simulink model "Drone_swarm_control"  (R2025a)
settings: Solver=FixedStepAuto  StartTime=0.0  StopTime=180  FixedStep=0.001  RelTol=1e-3
InitFcn:
  | %% Simulation parameters and waypoint trajectory
  | % Initial drone positions.
  | init_0=[0;0;0];
  | d_s=4;
  | init_1=init_0+d_s*[-1.1;0.1;0];
  | init_2=init_0+d_s*[0.3;-1.5;0];
  | init_3=init_0+d_s*[1.6;0.4;0];
  | init_4=init_0+d_s*[0.2;1.8;0];
  | 
  | % Initial battery energy in Wh.
  | E_0=77;
  | gain_2=1;
  | 
  | % PID controller gains.
  | PID_p=20;
  | PID_i=50;
  | PID_d=0;
  | 
  | % Router queues and background traffic.
  | router_buffer=160;
  | router_bandwith=300;
  | router_init_queue=[20,0,0,0,0];
  | traffic_mean=20;
  | traffic_variance=1;
  | 
  | % Communication-rate parameters.
  | F_max=2;
  | F_min=0.5;
  | F_H=(F_max+F_min)/3;
  | P_nc=(1-(F_H-F_min)/F_max);
  | 
  | 
  | % Desired formation offsets.
  | init_f_0=[0;0;0];
  | d_f=10;
  | init_f_1=init_0+d_f*[-1;0;0];
  | init_f_2=init_0+d_f*[0;-1;0];
  | init_f_3=init_0+d_f*[1;0;0];
  | init_f_4=init_0+d_f*[0;1;0];
  | 
  | 
  | % Waypoint mission with a fixed cruise altitude.
  | quota_fissa = -20;
  | 
  | waypoints = [
  |       0   0   0   0;
  |      75   0   quota_fissa   0;
  |     150   0   quota_fissa   0;
  |     225   0   quota_fissa   0;
  |     300   0   quota_fissa   0;
  |     300   0   quota_fissa   0;
  |     225  75   quota_fissa   0;
  |     150 150   quota_fissa   0;
  |      75 225   quota_fissa   0;
  |       0 300   quota_fissa   0;
  |       0 300   quota_fissa   0;
  |      75 300   quota_fissa   0;
  |     150 300   quota_fissa   0;
  |     225 300   quota_fissa   0;
  |     300 300   quota_fissa   0;
  | ... (+79 lines)
undefined symbols (not defined in the file): A_diacenza, DiscIntNeverNeededParam, L
libraries: dspsigops x10, robotcorelib x5, slpidlib x5, dspstat3 x5, simulink x1, uavutilslib x1
(part 2 of 4)

== system Drone_swarm_control/Subsystem1/Subsystem2 ==
  In1 : Inport
  In2 : Inport  Port=2
  In3 : Inport  Port=3
  In4 : Inport  Port=4
  In5 : Inport  Port=5
  Matrix Concatenate1 : Concatenate  NumInputs=5  Mode=Multidimensional array  ConcatenateDimension=2
  Out1 : Outport
  wires:
  In4/1 -> Matrix Concatenate1/4
  In2/1 -> Matrix Concatenate1/2
  In5/1 -> Matrix Concatenate1/5
  Matrix Concatenate1/1 -> Out1/1
  In1/1 -> Matrix Concatenate1/1
  In3/1 -> Matrix Concatenate1/3

== system Drone_swarm_control/Subsystem1/Subsystem3 ==
  In1 : Inport
  In2 : Inport  Port=2
  In3 : Inport  Port=3
  In4 : Inport  Port=4
  In5 : Inport  Port=5
  Matrix Concatenate3 : Concatenate  NumInputs=5  Mode=Multidimensional array  ConcatenateDimension=2
  Out1 : Outport
  wires:
  In5/1 -> Matrix Concatenate3/5
  Matrix Concatenate3/1 -> Out1/1
  In3/1 -> Matrix Concatenate3/3
  In4/1 -> Matrix Concatenate3/4
  In2/1 -> Matrix Concatenate3/2
  In1/1 -> Matrix Concatenate3/1

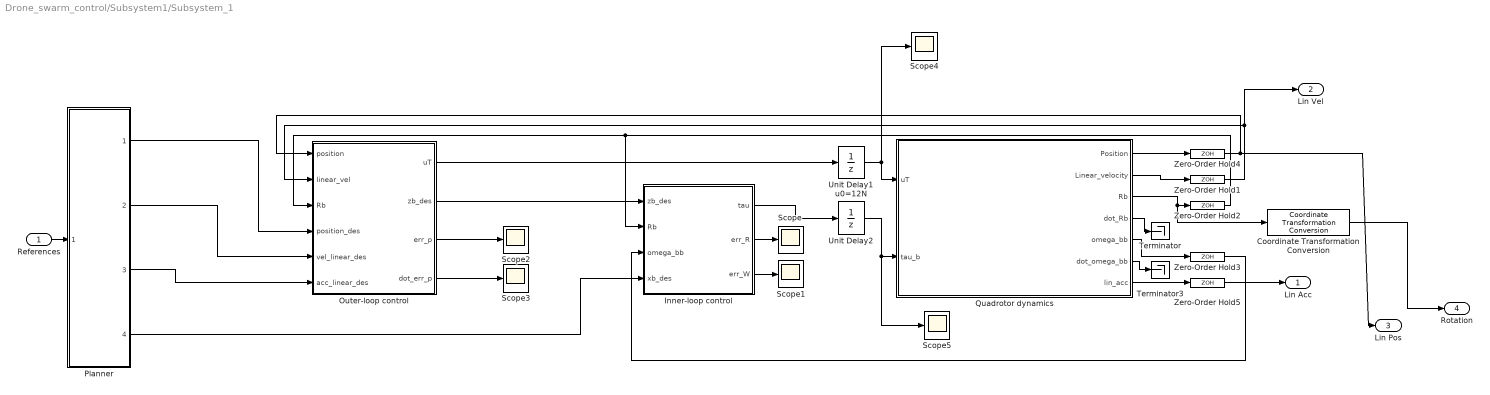
== system Drone_swarm_control/Subsystem1/Subsystem_1 ==
  References : Inport
  Coordinate Transformation Conversion : robotcorelib/Coordinate Transformation Conversion  InputRepresentation=Rotation Matrix  InputEulerSequence=ZYX  ShowTrVecInputPort=on  OutputRepresentation=Quaternion  OutputEulerSequence=ZYX  ShowTrVecOutputPort=on  SimulateUsing=Interpreted execution
  Inner-loop control : Subsystem
  Outer-loop control : MATLAB Function  TreatAsAtomicUnit=on
  Planner : Subsystem
  Quadrotor dynamics : Subsystem
  Scope{,1..5} (6 alike) : Scope
      Scope settings: ActiveDisplayYMinimum=-1.2E-5  ActiveDisplayYMaximum=1.2E-5
      Scope1 settings: ActiveDisplayYMinimum=-1.2E-5  ActiveDisplayYMaximum=1.2E-5
      Scope2 settings: ActiveDisplayYMinimum=-3.9E-5  ActiveDisplayYMaximum=1.1E-5  DataLoggingVariableName=ScopeData2
      Scope3 settings: ActiveDisplayYMinimum=-0.00022  ActiveDisplayYMaximum=0.00011  DataLoggingVariableName=ScopeData3
      Scope4 settings: ActiveDisplayYMinimum=11.66748  ActiveDisplayYMaximum=12.03695  DataLoggingVariableName=ScopeData4
      Scope5 settings: ActiveDisplayYMinimum=-0.02035  ActiveDisplayYMaximum=0.02036  DataLoggingVariableName=ScopeData5
  Terminator : Terminator
  Terminator3 : Terminator
  Unit Delay1 u0=12N : UnitDelay  InitialCondition=12  SampleTime=Ts
  Unit Delay2 : UnitDelay  InitialCondition=[0 0 0]  SampleTime=Ts
  Zero-Order Hold{1..5} (5 alike) : ZeroOrderHold  SampleTime=Ts
  Lin Acc : Outport
  Lin Vel : Outport  Port=2
  Lin Pos : Outport  Port=3
  Rotation : Outport  Port=4
  wires:
  Zero-Order Hold5/1 -> Lin Acc/1
  Quadrotor dynamics/7(lin_acc) -> Zero-Order Hold5/1
  Planner/1(position_des) -> Outer-loop control/4(position_des)
  Quadrotor dynamics/1(Position) -> Zero-Order Hold4/1
  Quadrotor dynamics/3(Rb) -> Zero-Order Hold2/1, Coordinate Transformation Conversion/1
  Quadrotor dynamics/4(dot_Rb) -> Terminator/1
  Planner/4(xb_des) -> Inner-loop control/4(xb_des)
  Inner-loop control/1(tau) -> Unit Delay2/1
  Planner/2(linear_velocity_des) -> Outer-loop control/5(vel_linear_des)
  Quadrotor dynamics/2(Linear_velocity) -> Zero-Order Hold1/1
  Quadrotor dynamics/6(dot_omega_bb) -> Terminator3/1
  Outer-loop control/3(err_p) -> Scope2/1
  Coordinate Transformation Conversion/1 -> Rotation/1
  Quadrotor dynamics/5(omega_bb) -> Zero-Order Hold3/1
  Zero-Order Hold2/1 -> Inner-loop control/2(Rb), Outer-loop control/3(Rb)
  References/1 -> Planner/1(References)
  Planner/3(linear_acceleration_des) -> Outer-loop control/6(acc_linear_des)
  Inner-loop control/3(err_W) -> Scope1/1
  Outer-loop control/2(zb_des) -> Inner-loop control/1(zb_des)
  Inner-loop control/2(err_R) -> Scope/1
  Outer-loop control/1(uT) -> Unit Delay1 u0=12N/1
  Unit Delay2/1 -> Quadrotor dynamics/2(tau_b), Scope5/1
  Zero-Order Hold3/1 -> Inner-loop control/3(omega_bb)
  Unit Delay1 u0=12N/1 -> Scope4/1, Quadrotor dynamics/1(uT)
  Outer-loop control/4(dot_err_p) -> Scope3/1
  Zero-Order Hold1/1 -> Outer-loop control/2(linear_vel), Lin Vel/1
  Zero-Order Hold4/1 -> Outer-loop control/1(position), Lin Pos/1

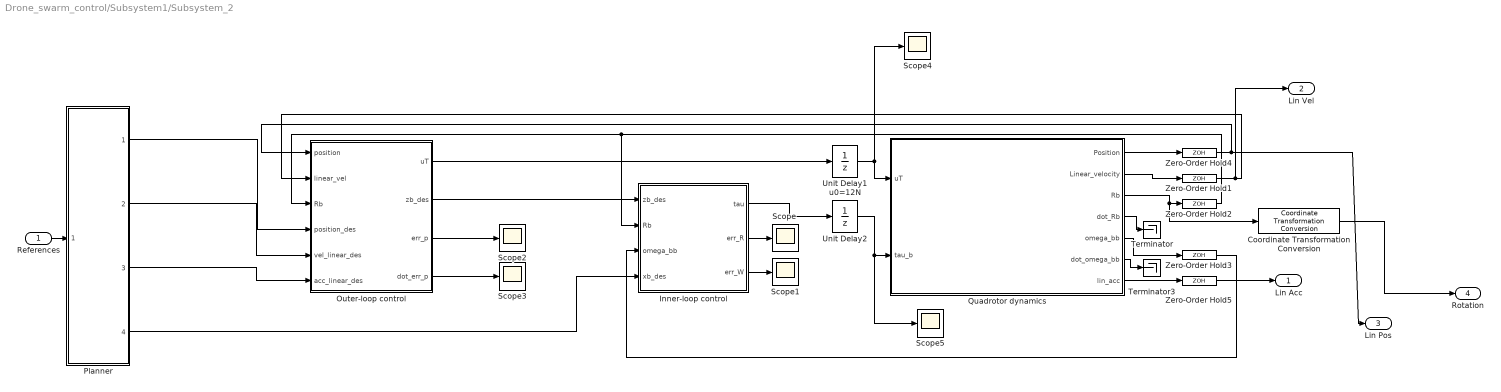
== system Drone_swarm_control/Subsystem1/Subsystem_2 ==
  References : Inport
  Coordinate Transformation Conversion : robotcorelib/Coordinate Transformation Conversion  InputRepresentation=Rotation Matrix  InputEulerSequence=ZYX  ShowTrVecInputPort=on  OutputRepresentation=Quaternion  OutputEulerSequence=ZYX  ShowTrVecOutputPort=on  SimulateUsing=Interpreted execution
  Inner-loop control : Subsystem
  Outer-loop control : MATLAB Function  TreatAsAtomicUnit=on
  Planner : Subsystem
  Quadrotor dynamics : Subsystem
  Scope{,1..5} (6 alike) : Scope
      Scope settings: ActiveDisplayYMinimum=-1.2E-5  ActiveDisplayYMaximum=1.2E-5
      Scope1 settings: ActiveDisplayYMinimum=-1.2E-5  ActiveDisplayYMaximum=1.2E-5
      Scope2 settings: ActiveDisplayYMinimum=-3.9E-5  ActiveDisplayYMaximum=1.1E-5  DataLoggingVariableName=ScopeData2
      Scope3 settings: ActiveDisplayYMinimum=-0.00022  ActiveDisplayYMaximum=0.00011  DataLoggingVariableName=ScopeData3
      Scope4 settings: ActiveDisplayYMinimum=11.66748  ActiveDisplayYMaximum=12.03695  DataLoggingVariableName=ScopeData4
      Scope5 settings: ActiveDisplayYMinimum=-0.02035  ActiveDisplayYMaximum=0.02036  DataLoggingVariableName=ScopeData5
  Terminator : Terminator
  Terminator3 : Terminator
  Unit Delay1 u0=12N : UnitDelay  InitialCondition=12  SampleTime=Ts
  Unit Delay2 : UnitDelay  InitialCondition=[0 0 0]  SampleTime=Ts
  Zero-Order Hold{1..5} (5 alike) : ZeroOrderHold  SampleTime=Ts
  Lin Acc : Outport
  Lin Vel : Outport  Port=2
  Lin Pos : Outport  Port=3
  Rotation : Outport  Port=4
  wires:
  Zero-Order Hold5/1 -> Lin Acc/1
  Quadrotor dynamics/7(lin_acc) -> Zero-Order Hold5/1
  Planner/1(position_des) -> Outer-loop control/4(position_des)
  Quadrotor dynamics/1(Position) -> Zero-Order Hold4/1
  Quadrotor dynamics/3(Rb) -> Zero-Order Hold2/1, Coordinate Transformation Conversion/1
  Quadrotor dynamics/4(dot_Rb) -> Terminator/1
  Planner/4(xb_des) -> Inner-loop control/4(xb_des)
  Inner-loop control/1(tau) -> Unit Delay2/1
  Planner/2(linear_velocity_des) -> Outer-loop control/5(vel_linear_des)
  Quadrotor dynamics/2(Linear_velocity) -> Zero-Order Hold1/1
  Quadrotor dynamics/6(dot_omega_bb) -> Terminator3/1
  Outer-loop control/3(err_p) -> Scope2/1
  Coordinate Transformation Conversion/1 -> Rotation/1
  Quadrotor dynamics/5(omega_bb) -> Zero-Order Hold3/1
  Zero-Order Hold2/1 -> Inner-loop control/2(Rb), Outer-loop control/3(Rb)
  References/1 -> Planner/1(References)
  Planner/3(linear_acceleration_des) -> Outer-loop control/6(acc_linear_des)
  Inner-loop control/3(err_W) -> Scope1/1
  Outer-loop control/2(zb_des) -> Inner-loop control/1(zb_des)
  Inner-loop control/2(err_R) -> Scope/1
  Outer-loop control/1(uT) -> Unit Delay1 u0=12N/1
  Unit Delay2/1 -> Quadrotor dynamics/2(tau_b), Scope5/1
  Zero-Order Hold3/1 -> Inner-loop control/3(omega_bb)
  Unit Delay1 u0=12N/1 -> Scope4/1, Quadrotor dynamics/1(uT)
  Outer-loop control/4(dot_err_p) -> Scope3/1
  Zero-Order Hold1/1 -> Outer-loop control/2(linear_vel), Lin Vel/1
  Zero-Order Hold4/1 -> Outer-loop control/1(position), Lin Pos/1

== system Drone_swarm_control/Subsystem1/Subsystem_3 ==
  References : Inport
  Coordinate Transformation Conversion : robotcorelib/Coordinate Transformation Conversion  InputRepresentation=Rotation Matrix  InputEulerSequence=ZYX  ShowTrVecInputPort=on  OutputRepresentation=Quaternion  OutputEulerSequence=ZYX  ShowTrVecOutputPort=on  SimulateUsing=Interpreted execution
  Inner-loop control : Subsystem
  Outer-loop control : MATLAB Function  TreatAsAtomicUnit=on
  Planner : Subsystem
  Quadrotor dynamics : Subsystem
  Scope{,1..5} (6 alike) : Scope
      Scope settings: ActiveDisplayYMinimum=-1.2E-5  ActiveDisplayYMaximum=1.2E-5
      Scope1 settings: ActiveDisplayYMinimum=-1.2E-5  ActiveDisplayYMaximum=1.2E-5
      Scope2 settings: ActiveDisplayYMinimum=-3.9E-5  ActiveDisplayYMaximum=1.1E-5  DataLoggingVariableName=ScopeData2
      Scope3 settings: ActiveDisplayYMinimum=-0.00022  ActiveDisplayYMaximum=0.00011  DataLoggingVariableName=ScopeData3
      Scope4 settings: ActiveDisplayYMinimum=11.66748  ActiveDisplayYMaximum=12.03695  DataLoggingVariableName=ScopeData4
      Scope5 settings: ActiveDisplayYMinimum=-0.02035  ActiveDisplayYMaximum=0.02036  DataLoggingVariableName=ScopeData5
  Terminator : Terminator
  Terminator3 : Terminator
  Unit Delay1 u0=12N : UnitDelay  InitialCondition=12  SampleTime=Ts
  Unit Delay2 : UnitDelay  InitialCondition=[0 0 0]  SampleTime=Ts
  Zero-Order Hold{1..5} (5 alike) : ZeroOrderHold  SampleTime=Ts
  Lin Acc : Outport
  Lin Vel : Outport  Port=2
  Lin Pos : Outport  Port=3
  Rotation : Outport  Port=4
  wires:
  Zero-Order Hold5/1 -> Lin Acc/1
  Quadrotor dynamics/7(lin_acc) -> Zero-Order Hold5/1
  Planner/1(position_des) -> Outer-loop control/4(position_des)
  Quadrotor dynamics/1(Position) -> Zero-Order Hold4/1
  Quadrotor dynamics/3(Rb) -> Zero-Order Hold2/1, Coordinate Transformation Conversion/1
  Quadrotor dynamics/4(dot_Rb) -> Terminator/1
  Planner/4(xb_des) -> Inner-loop control/4(xb_des)
  Inner-loop control/1(tau) -> Unit Delay2/1
  Planner/2(linear_velocity_des) -> Outer-loop control/5(vel_linear_des)
  Quadrotor dynamics/2(Linear_velocity) -> Zero-Order Hold1/1
  Quadrotor dynamics/6(dot_omega_bb) -> Terminator3/1
  Outer-loop control/3(err_p) -> Scope2/1
  Coordinate Transformation Conversion/1 -> Rotation/1
  Quadrotor dynamics/5(omega_bb) -> Zero-Order Hold3/1
  Zero-Order Hold2/1 -> Inner-loop control/2(Rb), Outer-loop control/3(Rb)
  References/1 -> Planner/1(References)
  Planner/3(linear_acceleration_des) -> Outer-loop control/6(acc_linear_des)
  Inner-loop control/3(err_W) -> Scope1/1
  Outer-loop control/2(zb_des) -> Inner-loop control/1(zb_des)
  Inner-loop control/2(err_R) -> Scope/1
  Outer-loop control/1(uT) -> Unit Delay1 u0=12N/1
  Unit Delay2/1 -> Quadrotor dynamics/2(tau_b), Scope5/1
  Zero-Order Hold3/1 -> Inner-loop control/3(omega_bb)
  Unit Delay1 u0=12N/1 -> Scope4/1, Quadrotor dynamics/1(uT)
  Outer-loop control/4(dot_err_p) -> Scope3/1
  Zero-Order Hold1/1 -> Outer-loop control/2(linear_vel), Lin Vel/1
  Zero-Order Hold4/1 -> Outer-loop control/1(position), Lin Pos/1

== system Drone_swarm_control/Subsystem1/Subsystem_4 ==
  References : Inport
  Coordinate Transformation Conversion : robotcorelib/Coordinate Transformation Conversion  InputRepresentation=Rotation Matrix  InputEulerSequence=ZYX  ShowTrVecInputPort=on  OutputRepresentation=Quaternion  OutputEulerSequence=ZYX  ShowTrVecOutputPort=on  SimulateUsing=Interpreted execution
  Inner-loop control : Subsystem
  Outer-loop control : MATLAB Function  TreatAsAtomicUnit=on
  Planner : Subsystem
  Quadrotor dynamics : Subsystem
  Scope{,1..5} (6 alike) : Scope
      Scope settings: ActiveDisplayYMinimum=-1.2E-5  ActiveDisplayYMaximum=1.2E-5
      Scope1 settings: ActiveDisplayYMinimum=-1.2E-5  ActiveDisplayYMaximum=1.2E-5
      Scope2 settings: ActiveDisplayYMinimum=-3.9E-5  ActiveDisplayYMaximum=1.1E-5  DataLoggingVariableName=ScopeData2
      Scope3 settings: ActiveDisplayYMinimum=-0.00022  ActiveDisplayYMaximum=0.00011  DataLoggingVariableName=ScopeData3
      Scope4 settings: ActiveDisplayYMinimum=11.66748  ActiveDisplayYMaximum=12.03695  DataLoggingVariableName=ScopeData4
      Scope5 settings: ActiveDisplayYMinimum=-0.02035  ActiveDisplayYMaximum=0.02036  DataLoggingVariableName=ScopeData5
  Terminator : Terminator
  Terminator3 : Terminator
  Unit Delay1 u0=12N : UnitDelay  InitialCondition=12  SampleTime=Ts
  Unit Delay2 : UnitDelay  InitialCondition=[0 0 0]  SampleTime=Ts
  Zero-Order Hold{1..5} (5 alike) : ZeroOrderHold  SampleTime=Ts
  Lin Acc : Outport
  Lin Vel : Outport  Port=2
  Lin Pos : Outport  Port=3
  Rotation : Outport  Port=4
  wires:
  Zero-Order Hold5/1 -> Lin Acc/1
  Quadrotor dynamics/7(lin_acc) -> Zero-Order Hold5/1
  Planner/1(position_des) -> Outer-loop control/4(position_des)
  Quadrotor dynamics/1(Position) -> Zero-Order Hold4/1
  Quadrotor dynamics/3(Rb) -> Zero-Order Hold2/1, Coordinate Transformation Conversion/1
  Quadrotor dynamics/4(dot_Rb) -> Terminator/1
  Planner/4(xb_des) -> Inner-loop control/4(xb_des)
  Inner-loop control/1(tau) -> Unit Delay2/1
  Planner/2(linear_velocity_des) -> Outer-loop control/5(vel_linear_des)
  Quadrotor dynamics/2(Linear_velocity) -> Zero-Order Hold1/1
  Quadrotor dynamics/6(dot_omega_bb) -> Terminator3/1
  Outer-loop control/3(err_p) -> Scope2/1
  Coordinate Transformation Conversion/1 -> Rotation/1
  Quadrotor dynamics/5(omega_bb) -> Zero-Order Hold3/1
  Zero-Order Hold2/1 -> Inner-loop control/2(Rb), Outer-loop control/3(Rb)
  References/1 -> Planner/1(References)
  Planner/3(linear_acceleration_des) -> Outer-loop control/6(acc_linear_des)
  Inner-loop control/3(err_W) -> Scope1/1
  Outer-loop control/2(zb_des) -> Inner-loop control/1(zb_des)
  Inner-loop control/2(err_R) -> Scope/1
  Outer-loop control/1(uT) -> Unit Delay1 u0=12N/1
  Unit Delay2/1 -> Quadrotor dynamics/2(tau_b), Scope5/1
  Zero-Order Hold3/1 -> Inner-loop control/3(omega_bb)
  Unit Delay1 u0=12N/1 -> Scope4/1, Quadrotor dynamics/1(uT)
  Outer-loop control/4(dot_err_p) -> Scope3/1
  Zero-Order Hold1/1 -> Outer-loop control/2(linear_vel), Lin Vel/1
  Zero-Order Hold4/1 -> Outer-loop control/1(position), Lin Pos/1

== system Drone_swarm_control/Subsystem1/Subsystem_5 ==
  References : Inport
  Coordinate Transformation Conversion : robotcorelib/Coordinate Transformation Conversion  InputRepresentation=Rotation Matrix  InputEulerSequence=ZYX  ShowTrVecInputPort=on  OutputRepresentation=Quaternion  OutputEulerSequence=ZYX  ShowTrVecOutputPort=on  SimulateUsing=Interpreted execution
  Inner-loop control : Subsystem
  Outer-loop control : MATLAB Function  TreatAsAtomicUnit=on
  Planner : Subsystem
  Quadrotor dynamics : Subsystem
  Scope{,1..5} (6 alike) : Scope
      Scope settings: ActiveDisplayYMinimum=-1.2E-5  ActiveDisplayYMaximum=1.2E-5
      Scope1 settings: ActiveDisplayYMinimum=-1.2E-5  ActiveDisplayYMaximum=1.2E-5
      Scope2 settings: ActiveDisplayYMinimum=-3.9E-5  ActiveDisplayYMaximum=1.1E-5  DataLoggingVariableName=ScopeData2
      Scope3 settings: ActiveDisplayYMinimum=-0.00022  ActiveDisplayYMaximum=0.00011  DataLoggingVariableName=ScopeData3
      Scope4 settings: ActiveDisplayYMinimum=11.66748  ActiveDisplayYMaximum=12.03695  DataLoggingVariableName=ScopeData4
      Scope5 settings: ActiveDisplayYMinimum=-0.02035  ActiveDisplayYMaximum=0.02036  DataLoggingVariableName=ScopeData5
  Terminator : Terminator
  Terminator3 : Terminator
  Unit Delay1 u0=12N : UnitDelay  InitialCondition=12  SampleTime=Ts
  Unit Delay2 : UnitDelay  InitialCondition=[0 0 0]  SampleTime=Ts
  Zero-Order Hold{1..5} (5 alike) : ZeroOrderHold  SampleTime=Ts
  Lin Acc : Outport
  Lin Vel : Outport  Port=2
  Lin Pos : Outport  Port=3
  Rotation : Outport  Port=4
  wires:
  Zero-Order Hold5/1 -> Lin Acc/1
  Quadrotor dynamics/7(lin_acc) -> Zero-Order Hold5/1
  Planner/1(position_des) -> Outer-loop control/4(position_des)
  Quadrotor dynamics/1(Position) -> Zero-Order Hold4/1
  Quadrotor dynamics/3(Rb) -> Zero-Order Hold2/1, Coordinate Transformation Conversion/1
  Quadrotor dynamics/4(dot_Rb) -> Terminator/1
  Planner/4(xb_des) -> Inner-loop control/4(xb_des)
  Inner-loop control/1(tau) -> Unit Delay2/1
  Planner/2(linear_velocity_des) -> Outer-loop control/5(vel_linear_des)
  Quadrotor dynamics/2(Linear_velocity) -> Zero-Order Hold1/1
  Quadrotor dynamics/6(dot_omega_bb) -> Terminator3/1
  Outer-loop control/3(err_p) -> Scope2/1
  Coordinate Transformation Conversion/1 -> Rotation/1
  Quadrotor dynamics/5(omega_bb) -> Zero-Order Hold3/1
  Zero-Order Hold2/1 -> Inner-loop control/2(Rb), Outer-loop control/3(Rb)
  References/1 -> Planner/1(References)
  Planner/3(linear_acceleration_des) -> Outer-loop control/6(acc_linear_des)
  Inner-loop control/3(err_W) -> Scope1/1
  Outer-loop control/2(zb_des) -> Inner-loop control/1(zb_des)
  Inner-loop control/2(err_R) -> Scope/1
  Outer-loop control/1(uT) -> Unit Delay1 u0=12N/1
  Unit Delay2/1 -> Quadrotor dynamics/2(tau_b), Scope5/1
  Zero-Order Hold3/1 -> Inner-loop control/3(omega_bb)
  Unit Delay1 u0=12N/1 -> Scope4/1, Quadrotor dynamics/1(uT)
  Outer-loop control/4(dot_err_p) -> Scope3/1
  Zero-Order Hold1/1 -> Outer-loop control/2(linear_vel), Lin Vel/1
  Zero-Order Hold4/1 -> Outer-loop control/1(position), Lin Pos/1

== system Drone_swarm_control/Subsystem13/Planner ==
  Constant : Constant  Value=0
  Mux{1..4} (4 alike) : Mux  Inputs=3
  Trigonometric Function : Trigonometry
  Trigonometric Function1 : Trigonometry  Operator=cos
  ddot_x_d : FromWorkspace  VariableName=[t' ddot_csi_d(1,:)']  SampleTime=Ts
  ddot_y_d : FromWorkspace  VariableName=[t' ddot_csi_d(2,:)']  SampleTime=Ts
  ddot_z_d : FromWorkspace  VariableName=[t' ddot_csi_d(3,:)']  SampleTime=Ts
  dot_x_d1 : FromWorkspace  VariableName=[t' dot_csi_d(1,:)']  SampleTime=Ts
  dot_y_d1 : FromWorkspace  VariableName=[t' dot_csi_d(2,:)']  SampleTime=Ts
  dot_z_d1 : FromWorkspace  VariableName=[t' dot_csi_d(3,:)']  SampleTime=Ts
  psi_d1 : FromWorkspace  VariableName=[t' psi_d']  SampleTime=Ts
  x_d : FromWorkspace  VariableName=[t' csi_d(1,:)']  SampleTime=Ts
  y_d : FromWorkspace  VariableName=[t' csi_d(2,:)']  SampleTime=Ts
  z_d : FromWorkspace  VariableName=[t' csi_d(3,:)']  SampleTime=Ts
  position_des : Outport
  linear_velocity_des : Outport  Port=2
  linear_acceleration_des : Outport  Port=3
  xb_des : Outport  Port=4
  wires:
  y_d/1 -> Mux1/2
  z_d/1 -> Mux1/3
  x_d/1 -> Mux1/1
  ddot_y_d/1 -> Mux2/2
  ddot_z_d/1 -> Mux2/3
  ddot_x_d/1 -> Mux2/1
  Mux2/1 -> linear_acceleration_des/1
  Mux1/1 -> position_des/1
  dot_y_d1/1 -> Mux3/2
  dot_z_d1/1 -> Mux3/3
  dot_x_d1/1 -> Mux3/1
  Mux3/1 -> linear_velocity_des/1
  Mux4/1 -> xb_des/1
  Trigonometric Function/1 -> Mux4/2
  psi_d1/1 -> Trigonometric Function/1, Trigonometric Function1/1
  Trigonometric Function1/1 -> Mux4/1
  Constant/1 -> Mux4/3

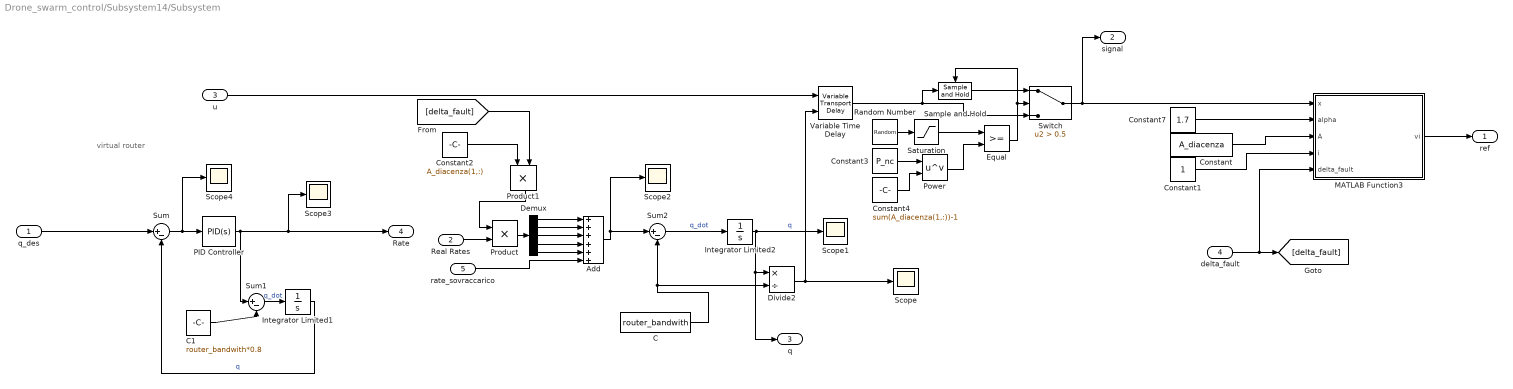
== system Drone_swarm_control/Subsystem14/Subsystem ==
  note: virtual router
  q_des : Inport
  " Real Rates" : Inport  Port=2
  u : Inport  Port=3
  delta_fault : Inport  Port=4
  "rate_sovraccarico " : Inport  Port=5
  Add : Sum  Inputs=++++++
  C : Constant  Value=router_bandwith
  C1 : Constant  Value=router_bandwith*0.8
  Constant : Constant  Value=A_diacenza
  Constant1 : Constant
  Constant2 : Constant  Value=A_diacenza(1,:)
  Constant3 : Constant  Value=P_nc
  Constant4 : Constant  Value=sum(A_diacenza(1,:))-1
  Constant7 : Constant  Value=1.7
  Demux : Demux  Outputs=5
  Divide2 : Product  Inputs=*/
  Equal : RelationalOperator  OutDataTypeStr=boolean  RndMeth=Simplest  InputSameDT=off
  Integrator Limited1 : Integrator  InitialCondition=router_init_queue(1)  LimitOutput=on  UpperSaturationLimit=router_buffer  LowerSaturationLimit=0
  Integrator Limited2 : Integrator  InitialCondition=router_init_queue(1)  LimitOutput=on  UpperSaturationLimit=router_buffer  LowerSaturationLimit=0
  MATLAB Function3 : MATLAB Function  TreatAsAtomicUnit=on
  PID Controller : slpidlib/PID Controller  Controller=PID  Form=Parallel  TimeDomain=Continuous-time  UseExternalTs=off  SampleTime=-1  IntegratorMethod=Forward Euler  FilterMethod=Forward Euler  ControllerParametersSource=internal  P=PID_p  I=PID_i  UseKiTs=off  D=PID_d  UseExternalDerivativeSource=off  N=100  UseFilter=on  TunerSelectOption=Transfer Function Based (PID Tuner App)  InitialConditionSource=internal  InitialConditionForIntegrator=0  InitialConditionForFilter=0  DifferentiatorICPrevScaledInput=0  ExternalReset=none  TrackingMode=off  Kt=1  LimitOutput=off  SatLimitsSource=internal  UpperSaturationLimit=inf  LowerSaturationLimit=-inf  LinearizeAsGain=on  AntiWindupMode=none  Kb=1  LimitIntegrator=off  UpperIntegratorSaturationLimit=inf  LowerIntegratorSaturationLimit=-inf  POutMin=[]  POutMax=[]  IOutMin=[]  IOutMax=[]  DOutMin=[]  DOutMax=[]  NOutMin=[]  NOutMax=[]  SumOutMin=[]  SumOutMax=[]  SaturationOutMin=[]  SaturationOutMax=[]  PParamMin=[]  PParamMax=[]  IParamMin=[]  IParamMax=[]  DParamMin=[]  DParamMax=[]  NParamMin=[]  NParamMax=[]  KbParamMin=[]  KbParamMax=[]  KtParamMin=[]  KtParamMax=[]  KbOutMin=[]  KbOutMax=[]  KtOutMin=[]  KtOutMax=[]  IntegratorOutMin=[]  IntegratorOutMax=[]  FilterOutMin=[]  FilterOutMax=[]  SumI1OutMin=[]  SumI1OutMax=[]  SumI2OutMin=[]  SumI2OutMax=[]  SumI3OutMin=[]  SumI3OutMax=[]  SumI4OutMin=[]  SumI4OutMax=[]  SumDOutMin=[]  SumDOutMax=[]  DifferentiatorOutMin=[]  DifferentiatorOutMax=[]  FilterDiffOutCoefMin=[]  FilterDiffOutCoefMax=[]  ReciprocalOutMin=[]  ReciprocalOutMax=[]  SumDenOutMin=[]  SumDenOutMax=[]  SumNumOutMin=[]  SumNumOutMax=[]  DivideOutMin=[]  DivideOutMax=[]  UdiffTsProdOutMin=[]  UdiffTsProdOutMax=[]  NTsProdOutMin=[]  NTsProdOutMax=[]  UintegralTsProdOutMin=[]  UintegralTsProdOutMax=[]  UngainTsProdOutMin=[]  UngainTsProdOutMax=[]  ClampingZeroOutDataTypeStr=Inherit: Inherit via back propagation  ClampingZeroOutMin=[]  ClampingZeroOutMax=[]  FilterDenConstantOutDataTypeStr=Inherit: Inherit via back propagation  FilterDenConstantOutMin=[]  FilterDenConstantOutMax=[]  PCopyOutDataTypeStr=Inherit: Inherit via back propagation  PCopyOutMin=[]  PCopyOutMax=[]  NCopyOutDataTypeStr=Inherit: Inherit via back propagation  NCopyOutMin=[]  NCopyOutMax=[]  IntegratorContinuousStateAttributes=''  IntegratorStateMustResolveToSignalObject=off  IntegratorRTWStateStorageClass=Auto  FilterContinuousStateAttributes=''  FilterStateMustResolveToSignalObject=off  FilterRTWStateStorageClass=Auto  ParallelPVariant=InternalParameters  IdealPVariant=Disabled  IVariant=InternalParameters  DVariant=InternalParameters  IntegratorVariant=Continuous  SatVariant=Disabled  AWVariant=Passthrough  PCopyVariant=Disabled  TRVariant=Disabled  FdbkBlocksVariant=Forward  IdealPFdbkVariant=Disabled  SatFdbkVariant=Disabled  DerivativeFilterVariant=ContFilter  NVariant=InternalParameters  NCopyVariant=Disabled  FilterICVariant=InternalICsFilter  IntegratorICVariant=InternalICs  ExternalResetVariant=Disabled  TRSumVariant=Passthrough  SumFdbkVariant=Disabled  SumVariant=Sum_PID  TsampFilterVariant=InternalTs  TsampNgainVariant=Passthrough  TsampIntegralVariant=Disabled_SignalSpec  ExternalSaturationOutDataTypeStr=Inherit: Same as second input  DerivativeSourceVariant=ErrorSignal  PreIntVariant=InternalPreInt
  Power : Math  Operator=pow
  Product : Product
  Product1 : Product
  Random Number : RandomNumber  Mean=0.5  Variance=0.5  SampleTime=0.1
  Sample and Hold : dspsigops/Sample and Hold  trig=Rising edge  initCond=0  latchinput=off
  Saturation : Saturate  UpperLimit=1  LowerLimit=0
  Scope{,1..4} (5 alike) : Scope
      Scope settings: ActiveDisplayYMinimum=-1  ActiveDisplayYMaximum=1  DataLoggingVariableName=ScopeData7
      Scope1 settings: ActiveDisplayYMinimum=-1  ActiveDisplayYMaximum=1  DataLoggingVariableName=ScopeData8
      Scope2 settings: ActiveDisplayYMinimum=-1  ActiveDisplayYMaximum=1  DataLoggingVariableName=ScopeData13
      Scope3 settings: ActiveDisplayYMinimum=18.031914924971169  ActiveDisplayYMaximum=21.223404282118214  DataLoggingVariableName=ScopeData12
      Scope4 settings: ActiveDisplayYMinimum=-3.625  ActiveDisplayYMaximum=2.625  DataLoggingVariableName=ScopeData29
  Sum : Sum  Inputs=|+-
  Sum1 : Sum  Inputs=|+-
  Sum2 : Sum  Inputs=|+-
  Switch : Switch  Criteria=u2 > Threshold  Threshold=0.5  SaturateOnIntegerOverflow=off  InputSameDT=off
  Variable Time Delay : VariableTransportDelay  MaximumDelay=1000  InitialOutput=[init_0;zeros(6,1);init_1;zeros(6,1);init_2;zeros(6,1);init_3;zeros(6,1);init_4;zeros(6,1);]  MaximumPoints=1e4  ZeroDelay=on
  ref : Outport
  "signal " : Outport  Port=2
  q : Outport  Port=3
  " Rate" : Outport  Port=4
  wires:
  Constant7/1 -> MATLAB Function3/2(alpha)
  Constant/1 -> MATLAB Function3/3(A)
  Constant1/1 -> MATLAB Function3/4(i)
  MATLAB Function3/1(vi) -> ref/1
  Integrator Limited2/1 -> q/1, Divide2/1, Scope1/1  "q"
  Switch/1 -> "signal "/1, MATLAB Function3/1(x)
  u/1 -> Variable Time Delay/1
  Sum2/1 -> Integrator Limited2/1  "q_dot"
  Divide2/1 -> Scope/1, Variable Time Delay/2
  C/1 -> Sum2/2, Divide2/2
  Variable Time Delay/1 -> Sample and Hold/1, Switch/3
  PID Controller/1 -> Sum1/1, " Rate"/1, Scope3/1
  Sum/1 -> Scope4/1, PID Controller/1
  q_des/1 -> Sum/1
  Sum1/1 -> Integrator Limited1/1  "q_dot"
  Integrator Limited1/1 -> Sum/2  "q"
  C1/1 -> Sum1/2
  Demux/3 -> Add/3
  Demux/4 -> Add/4
  Demux/2 -> Add/2
  Demux/5 -> Add/5
  Demux/1 -> Add/1
  Add/1 -> Scope2/1, Sum2/1
  " Real Rates"/1 -> Product/2
  Product/1 -> Demux/1
  Random Number/1 -> Saturation/1
  Equal/1 -> Sample and Hold/Trigger, Switch/2
  Power/1 -> Equal/2
  Saturation/1 -> Equal/1
  Constant3/1 -> Power/1
  Constant4/1 -> Power/2
  Sample and Hold/1 -> Switch/1
  delta_fault/1 -> [delta_fault], MATLAB Function3/5(delta_fault)
  Product1/1 -> Product/1
  Constant2/1 -> Product1/1
  [delta_fault] -> Product1/2
  "rate_sovraccarico "/1 -> Add/6

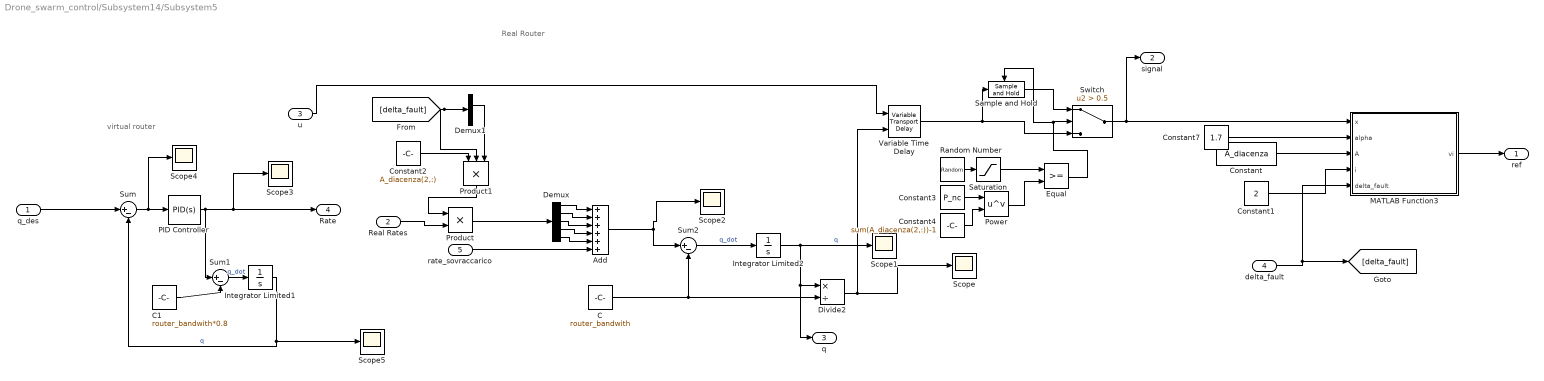
== system Drone_swarm_control/Subsystem14/Subsystem5 ==
  note: Real Router
  note: virtual router
  q_des : Inport
  " Real Rates" : Inport  Port=2
  u : Inport  Port=3
  delta_fault : Inport  Port=4
  "rate_sovraccarico " : Inport  Port=5
  Add : Sum  Inputs=++++++
  C : Constant  Value=router_bandwith
  C1 : Constant  Value=router_bandwith*0.8
  Constant : Constant  Value=A_diacenza
  Constant1 : Constant  Value=2
  Constant2 : Constant  Value=A_diacenza(2,:)
  Constant3 : Constant  Value=P_nc
  Constant4 : Constant  Value=sum(A_diacenza(2,:))-1
  Constant7 : Constant  Value=1.7
  Demux : Demux  Outputs=5
  Demux1 : Demux  Outputs=5
  Divide2 : Product  Inputs=*/
  Equal : RelationalOperator  OutDataTypeStr=boolean  RndMeth=Simplest  InputSameDT=off
  Integrator Limited1 : Integrator  InitialCondition=router_init_queue(1)  LimitOutput=on  UpperSaturationLimit=router_buffer  LowerSaturationLimit=0
  Integrator Limited2 : Integrator  InitialCondition=router_init_queue(2)  LimitOutput=on  UpperSaturationLimit=router_buffer  LowerSaturationLimit=0
  MATLAB Function3 : MATLAB Function  TreatAsAtomicUnit=on
  PID Controller : slpidlib/PID Controller  Controller=PID  Form=Parallel  TimeDomain=Continuous-time  UseExternalTs=off  SampleTime=-1  IntegratorMethod=Forward Euler  FilterMethod=Forward Euler  ControllerParametersSource=internal  P=PID_p  I=PID_i  UseKiTs=off  D=PID_d  UseExternalDerivativeSource=off  N=100  UseFilter=on  TunerSelectOption=Transfer Function Based (PID Tuner App)  InitialConditionSource=internal  InitialConditionForIntegrator=0  InitialConditionForFilter=0  DifferentiatorICPrevScaledInput=0  ExternalReset=none  TrackingMode=off  Kt=1  LimitOutput=off  SatLimitsSource=internal  UpperSaturationLimit=inf  LowerSaturationLimit=-inf  LinearizeAsGain=on  AntiWindupMode=none  Kb=1  LimitIntegrator=off  UpperIntegratorSaturationLimit=inf  LowerIntegratorSaturationLimit=-inf  POutMin=[]  POutMax=[]  IOutMin=[]  IOutMax=[]  DOutMin=[]  DOutMax=[]  NOutMin=[]  NOutMax=[]  SumOutMin=[]  SumOutMax=[]  SaturationOutMin=[]  SaturationOutMax=[]  PParamMin=[]  PParamMax=[]  IParamMin=[]  IParamMax=[]  DParamMin=[]  DParamMax=[]  NParamMin=[]  NParamMax=[]  KbParamMin=[]  KbParamMax=[]  KtParamMin=[]  KtParamMax=[]  KbOutMin=[]  KbOutMax=[]  KtOutMin=[]  KtOutMax=[]  IntegratorOutMin=[]  IntegratorOutMax=[]  FilterOutMin=[]  FilterOutMax=[]  SumI1OutMin=[]  SumI1OutMax=[]  SumI2OutMin=[]  SumI2OutMax=[]  SumI3OutMin=[]  SumI3OutMax=[]  SumI4OutMin=[]  SumI4OutMax=[]  SumDOutMin=[]  SumDOutMax=[]  DifferentiatorOutMin=[]  DifferentiatorOutMax=[]  FilterDiffOutCoefMin=[]  FilterDiffOutCoefMax=[]  ReciprocalOutMin=[]  ReciprocalOutMax=[]  SumDenOutMin=[]  SumDenOutMax=[]  SumNumOutMin=[]  SumNumOutMax=[]  DivideOutMin=[]  DivideOutMax=[]  UdiffTsProdOutMin=[]  UdiffTsProdOutMax=[]  NTsProdOutMin=[]  NTsProdOutMax=[]  UintegralTsProdOutMin=[]  UintegralTsProdOutMax=[]  UngainTsProdOutMin=[]  UngainTsProdOutMax=[]  ClampingZeroOutDataTypeStr=Inherit: Inherit via back propagation  ClampingZeroOutMin=[]  ClampingZeroOutMax=[]  FilterDenConstantOutDataTypeStr=Inherit: Inherit via back propagation  FilterDenConstantOutMin=[]  FilterDenConstantOutMax=[]  PCopyOutDataTypeStr=Inherit: Inherit via back propagation  PCopyOutMin=[]  PCopyOutMax=[]  NCopyOutDataTypeStr=Inherit: Inherit via back propagation  NCopyOutMin=[]  NCopyOutMax=[]  IntegratorContinuousStateAttributes=''  IntegratorStateMustResolveToSignalObject=off  IntegratorRTWStateStorageClass=Auto  FilterContinuousStateAttributes=''  FilterStateMustResolveToSignalObject=off  FilterRTWStateStorageClass=Auto  ParallelPVariant=InternalParameters  IdealPVariant=Disabled  IVariant=InternalParameters  DVariant=InternalParameters  IntegratorVariant=Continuous  SatVariant=Disabled  AWVariant=Passthrough  PCopyVariant=Disabled  TRVariant=Disabled  FdbkBlocksVariant=Forward  IdealPFdbkVariant=Disabled  SatFdbkVariant=Disabled  DerivativeFilterVariant=ContFilter  NVariant=InternalParameters  NCopyVariant=Disabled  FilterICVariant=InternalICsFilter  IntegratorICVariant=InternalICs  ExternalResetVariant=Disabled  TRSumVariant=Passthrough  SumFdbkVariant=Disabled  SumVariant=Sum_PID  TsampFilterVariant=InternalTs  TsampNgainVariant=Passthrough  TsampIntegralVariant=Disabled_SignalSpec  ExternalSaturationOutDataTypeStr=Inherit: Same as second input  DerivativeSourceVariant=ErrorSignal  PreIntVariant=InternalPreInt
  Power : Math  Operator=pow
  Product : Product
  Product1 : Product  Inputs=3
  Random Number : RandomNumber  Mean=0.5  Variance=0.5  SampleTime=0.1
  Sample and Hold : dspsigops/Sample and Hold  trig=Rising edge  initCond=0  latchinput=off
  Saturation : Saturate  UpperLimit=1  LowerLimit=0
  Scope{,1..5} (6 alike) : Scope
      Scope settings: DataLoggingVariableName=ScopeData7
      Scope1 settings: ActiveDisplayYMinimum=-1  ActiveDisplayYMaximum=1  DataLoggingVariableName=ScopeData8
      Scope2 settings: ActiveDisplayYMinimum=-4.9997275794883738  ActiveDisplayYMaximum=44.997548215395369  DataLoggingVariableName=ScopeData13
      Scope3 settings: ActiveDisplayYMinimum=-48.354575152001019  ActiveDisplayYMaximum=35.191176368009138  DataLoggingVariableName=ScopeData14
      Scope4 settings: ActiveDisplayYMinimum=-3.625  ActiveDisplayYMaximum=2.625  DataLoggingVariableName=ScopeData15
      Scope5 settings: ActiveDisplayYMinimum=-0.24999999999999994  ActiveDisplayYMaximum=2.25  DataLoggingVariableName=ScopeData25
  Sum : Sum  Inputs=|+-
  Sum1 : Sum  Inputs=|+-
  Sum2 : Sum  Inputs=|+-
  Switch : Switch  Criteria=u2 > Threshold  Threshold=0.5  SaturateOnIntegerOverflow=off  InputSameDT=off
  Variable Time Delay : VariableTransportDelay  MaximumDelay=1000  InitialOutput=[init_0;zeros(6,1);init_1;zeros(6,1);init_2;zeros(6,1);init_3;zeros(6,1);init_4;zeros(6,1);]  MaximumPoints=1e4  ZeroDelay=on
  ref : Outport
  "signal " : Outport  Port=2
  q : Outport  Port=3
  " Rate" : Outport  Port=4
  wires:
  Sample and Hold/1 -> Switch/1
  Variable Time Delay/1 -> Sample and Hold/1, Switch/3
  C/1 -> Sum2/2, Divide2/2
  Divide2/1 -> Variable Time Delay/2, Scope/1
  Sum2/1 -> Integrator Limited2/1  "q_dot"
  u/1 -> Variable Time Delay/1
  Switch/1 -> MATLAB Function3/1(x), "signal "/1
  Integrator Limited2/1 -> Divide2/1, q/1, Scope1/1  "q"
  MATLAB Function3/1(vi) -> ref/1
  Constant1/1 -> MATLAB Function3/4(i)
  Constant/1 -> MATLAB Function3/3(A)
  Constant7/1 -> MATLAB Function3/2(alpha)
  PID Controller/1 -> " Rate"/1, Scope3/1, Sum1/1
  q_des/1 -> Sum/1
  Sum1/1 -> Integrator Limited1/1  "q_dot"
  Sum/1 -> Scope4/1, PID Controller/1
  C1/1 -> Sum1/2
  Integrator Limited1/1 -> Scope5/1, Sum/2  "q"
  Demux/3 -> Add/3
  Demux/2 -> Add/2
  " Real Rates"/1 -> Product/2
  Demux/4 -> Add/4
  Demux/5 -> Add/5
  Demux/1 -> Add/1
  Product/1 -> Demux/1
  Add/1 -> Scope2/1, Sum2/1
  Power/1 -> Equal/2
  Saturation/1 -> Equal/1
  Constant3/1 -> Power/1
  Random Number/1 -> Saturation/1
  Constant4/1 -> Power/2
  Equal/1 -> Sample and Hold/Trigger, Switch/2
  Product1/1 -> Product/1
  [delta_fault] -> Product1/2, Demux1/1
  Constant2/1 -> Product1/1
  delta_fault/1 -> [delta_fault], MATLAB Function3/5(delta_fault)
  Demux1/2 -> Product1/3
  "rate_sovraccarico "/1 -> Add/6

== system Drone_swarm_control/Subsystem14/Subsystem7 ==
  q_ref : Inport
  " r_min" : Inport  Port=2
  u : Inport  Port=3
  delta_fault : Inport  Port=4
  "rate_sovraccarico " : Inport  Port=5
  Constant : Constant  Value=A_diacenza
  Constant1 : Constant  Value=3
  Constant7 : Constant  Value=1.7
  MATLAB Function3 : MATLAB Function  TreatAsAtomicUnit=on
  "Real Router " : Subsystem
      settings: PortSchema="{\"entries\":[{\"content\":{\"sides\":[{\"content\":{\"connectorIds\":[\"In1\",\"In2\",\"In3\"]},\"type\":\"ConnectorPlacement.EquallySpacedRectSide\",\"uuid\":\"e82b9b07-ca0e-408d-a443-8ff1c64233a8\"},{\"content\":{\"connectorIds\":[\"Out1\",\"Out2\"],\"side\":\"RIGHT\"},\"type\":\"ConnectorPlacement.EquallySpacedRectSide\",\"uuid\":\"b3c90e89-7809-413d-ba2c-0a4ea40c01e5\"},{\"content\":{\"side\":\"TOP\"},\"type\":\"ConnectorPlacement.EquallySpacedRectSide\",\"uuid\":\"7b654019-7638-4ba3-873e-3beda5d7f92f\"},{\"content\":{\"connectorIds\":[\"In4\"],\"side\":\"BOTTOM\"},\"type\":\"ConnectorPlacement.EquallySpacedRectSide\",\"uuid\":\"99466aa8-6c56-4521-a07d-3b5417d28f3d\"}]},\"type\":\"ConnectorPlacement.EquallySpacedConnector\",\"uuid\":\"eaa7be40-ee25-4428-a86e-d4fbbbf587ec\"}],\"packageUris\":[\"http://schema.mathworks.com/mf0/Connector/R2020b\"],\"version\":\"1.0\"}"
  virtual router : Subsystem
  ref : Outport
  "signal " : Outport  Port=2
  q : Outport  Port=3
  " r_req" : Outport  Port=4
  wires:
  Constant7/1 -> MATLAB Function3/2(alpha)
  Constant/1 -> MATLAB Function3/3(A)
  Constant1/1 -> MATLAB Function3/4(i)
  MATLAB Function3/1(vi) -> ref/1
  delta_fault/1 -> [delta_fault], MATLAB Function3/5(delta_fault)
  "Real Router "/1(state variables_out) -> MATLAB Function3/1(x), "signal "/1
  u/1 -> "Real Router "/1(state variables_in)
  [delta_fault] -> "Real Router "/2(delta_fault)
  " r_min"/1 -> "Real Router "/3(Real Rates)
  "Real Router "/2(q) -> q/1
  q_ref/1 -> virtual router/1(q_ref)
  virtual router/1(r_req) -> " r_req"/1
  "rate_sovraccarico "/1 -> "Real Router "/4("rate_sovraccarico ")

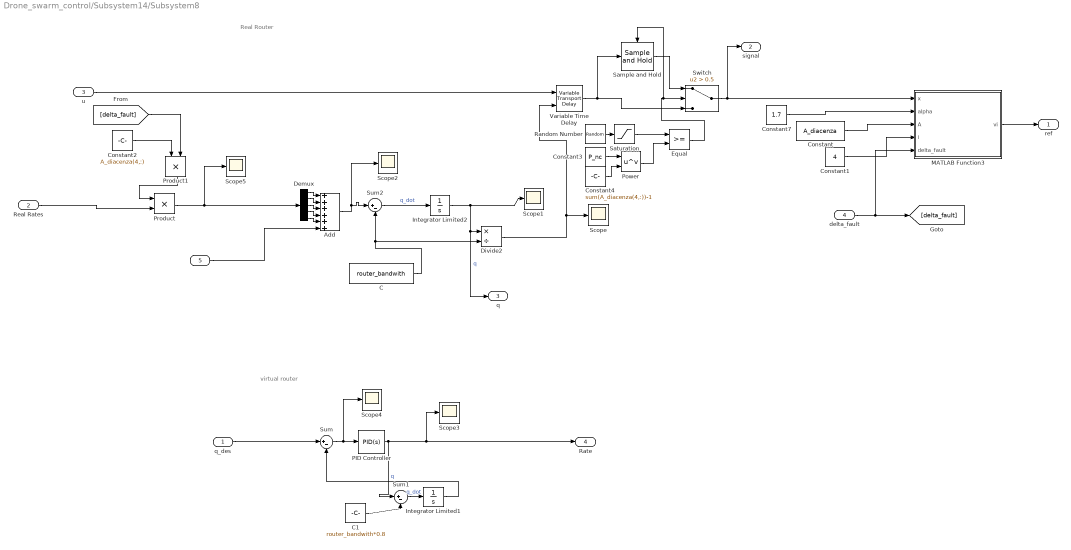
== system Drone_swarm_control/Subsystem14/Subsystem8 ==
  note: Real Router
  note: virtual router
  q_des : Inport
  " Real Rates" : Inport  Port=2
  u : Inport  Port=3
  delta_fault : Inport  Port=4
  " " : Inport  Port=5
  Add : Sum  Inputs=++++++
  C : Constant  Value=router_bandwith
  C1 : Constant  Value=router_bandwith*0.8
  Constant : Constant  Value=A_diacenza
  Constant1 : Constant  Value=4
  Constant2 : Constant  Value=A_diacenza(4,:)
  Constant3 : Constant  Value=P_nc
  Constant4 : Constant  Value=sum(A_diacenza(4,:))-1
  Constant7 : Constant  Value=1.7
  Demux : Demux  Outputs=5
  Divide2 : Product  Inputs=*/
  Equal : RelationalOperator  OutDataTypeStr=boolean  RndMeth=Simplest  InputSameDT=off
  Integrator Limited1 : Integrator  InitialCondition=router_init_queue(1)  LimitOutput=on  UpperSaturationLimit=router_buffer  LowerSaturationLimit=0
  Integrator Limited2 : Integrator  InitialCondition=router_init_queue(4)  LimitOutput=on  UpperSaturationLimit=router_buffer  LowerSaturationLimit=0
  MATLAB Function3 : MATLAB Function  TreatAsAtomicUnit=on
  PID Controller : slpidlib/PID Controller  Controller=PID  Form=Parallel  TimeDomain=Continuous-time  UseExternalTs=off  SampleTime=-1  IntegratorMethod=Forward Euler  FilterMethod=Forward Euler  ControllerParametersSource=internal  P=PID_p  I=PID_i  UseKiTs=off  D=PID_d  UseExternalDerivativeSource=off  N=100  UseFilter=on  TunerSelectOption=Transfer Function Based (PID Tuner App)  InitialConditionSource=internal  InitialConditionForIntegrator=0  InitialConditionForFilter=0  DifferentiatorICPrevScaledInput=0  ExternalReset=none  TrackingMode=off  Kt=1  LimitOutput=off  SatLimitsSource=internal  UpperSaturationLimit=inf  LowerSaturationLimit=-inf  LinearizeAsGain=on  AntiWindupMode=none  Kb=1  LimitIntegrator=off  UpperIntegratorSaturationLimit=inf  LowerIntegratorSaturationLimit=-inf  POutMin=[]  POutMax=[]  IOutMin=[]  IOutMax=[]  DOutMin=[]  DOutMax=[]  NOutMin=[]  NOutMax=[]  SumOutMin=[]  SumOutMax=[]  SaturationOutMin=[]  SaturationOutMax=[]  PParamMin=[]  PParamMax=[]  IParamMin=[]  IParamMax=[]  DParamMin=[]  DParamMax=[]  NParamMin=[]  NParamMax=[]  KbParamMin=[]  KbParamMax=[]  KtParamMin=[]  KtParamMax=[]  KbOutMin=[]  KbOutMax=[]  KtOutMin=[]  KtOutMax=[]  IntegratorOutMin=[]  IntegratorOutMax=[]  FilterOutMin=[]  FilterOutMax=[]  SumI1OutMin=[]  SumI1OutMax=[]  SumI2OutMin=[]  SumI2OutMax=[]  SumI3OutMin=[]  SumI3OutMax=[]  SumI4OutMin=[]  SumI4OutMax=[]  SumDOutMin=[]  SumDOutMax=[]  DifferentiatorOutMin=[]  DifferentiatorOutMax=[]  FilterDiffOutCoefMin=[]  FilterDiffOutCoefMax=[]  ReciprocalOutMin=[]  ReciprocalOutMax=[]  SumDenOutMin=[]  SumDenOutMax=[]  SumNumOutMin=[]  SumNumOutMax=[]  DivideOutMin=[]  DivideOutMax=[]  UdiffTsProdOutMin=[]  UdiffTsProdOutMax=[]  NTsProdOutMin=[]  NTsProdOutMax=[]  UintegralTsProdOutMin=[]  UintegralTsProdOutMax=[]  UngainTsProdOutMin=[]  UngainTsProdOutMax=[]  ClampingZeroOutDataTypeStr=Inherit: Inherit via back propagation  ClampingZeroOutMin=[]  ClampingZeroOutMax=[]  FilterDenConstantOutDataTypeStr=Inherit: Inherit via back propagation  FilterDenConstantOutMin=[]  FilterDenConstantOutMax=[]  PCopyOutDataTypeStr=Inherit: Inherit via back propagation  PCopyOutMin=[]  PCopyOutMax=[]  NCopyOutDataTypeStr=Inherit: Inherit via back propagation  NCopyOutMin=[]  NCopyOutMax=[]  IntegratorContinuousStateAttributes=''  IntegratorStateMustResolveToSignalObject=off  IntegratorRTWStateStorageClass=Auto  FilterContinuousStateAttributes=''  FilterStateMustResolveToSignalObject=off  FilterRTWStateStorageClass=Auto  ParallelPVariant=InternalParameters  IdealPVariant=Disabled  IVariant=InternalParameters  DVariant=InternalParameters  IntegratorVariant=Continuous  SatVariant=Disabled  AWVariant=Passthrough  PCopyVariant=Disabled  TRVariant=Disabled  FdbkBlocksVariant=Forward  IdealPFdbkVariant=Disabled  SatFdbkVariant=Disabled  DerivativeFilterVariant=ContFilter  NVariant=InternalParameters  NCopyVariant=Disabled  FilterICVariant=InternalICsFilter  IntegratorICVariant=InternalICs  ExternalResetVariant=Disabled  TRSumVariant=Passthrough  SumFdbkVariant=Disabled  SumVariant=Sum_PID  TsampFilterVariant=InternalTs  TsampNgainVariant=Passthrough  TsampIntegralVariant=Disabled_SignalSpec  ExternalSaturationOutDataTypeStr=Inherit: Same as second input  DerivativeSourceVariant=ErrorSignal  PreIntVariant=InternalPreInt
  Power : Math  Operator=pow
  Product : Product
  Product1 : Product
  Random Number : RandomNumber  Mean=0.5  Variance=0.5  SampleTime=0.1
  Sample and Hold : dspsigops/Sample and Hold  trig=Rising edge  initCond=0  latchinput=off
  Saturation : Saturate  UpperLimit=1  LowerLimit=0
  Scope{,1..5} (6 alike) : Scope
      Scope settings: DataLoggingVariableName=ScopeData7
      Scope1 settings: ActiveDisplayYMinimum=-1  ActiveDisplayYMaximum=1  DataLoggingVariableName=ScopeData8
      Scope2 settings: ActiveDisplayYMinimum=-16.4776588849588  ActiveDisplayYMaximum=28.850052227950371  DataLoggingVariableName=ScopeData13
      Scope3 settings: ActiveDisplayYMinimum=18.031914924971169  ActiveDisplayYMaximum=21.223404282118214  DataLoggingVariableName=ScopeData16
      Scope4 settings: ActiveDisplayYMinimum=-3.625  ActiveDisplayYMaximum=2.625  DataLoggingVariableName=ScopeData17
      Scope5 settings: ActiveDisplayYMinimum=-24.1772735307082  ActiveDisplayYMaximum=17.595461776373806  DataLoggingVariableName=ScopeData24
  Sum : Sum  Inputs=|+-
  Sum1 : Sum  Inputs=|+-
  Sum2 : Sum  Inputs=|+-
  Switch : Switch  Criteria=u2 > Threshold  Threshold=0.5  SaturateOnIntegerOverflow=off  InputSameDT=off
  Variable Time Delay : VariableTransportDelay  MaximumDelay=1000  InitialOutput=[init_0;zeros(6,1);init_1;zeros(6,1);init_2;zeros(6,1);init_3;zeros(6,1);init_4;zeros(6,1);]  MaximumPoints=1e4  ZeroDelay=on
  ref : Outport
  "signal " : Outport  Port=2
  q : Outport  Port=3
  " Rate" : Outport  Port=4
  wires:
  Sample and Hold/1 -> Switch/1
  Variable Time Delay/1 -> Sample and Hold/1, Switch/3
  C/1 -> Sum2/2, Divide2/2
  Divide2/1 -> Variable Time Delay/2, Scope/1
  Sum2/1 -> Integrator Limited2/1  "q_dot"
  u/1 -> Variable Time Delay/1
  Switch/1 -> MATLAB Function3/1(x), "signal "/1
  Integrator Limited2/1 -> Scope1/1, q/1, Divide2/1  "q"
  MATLAB Function3/1(vi) -> ref/1
  Constant1/1 -> MATLAB Function3/4(i)
  Constant/1 -> MATLAB Function3/3(A)
  Constant7/1 -> MATLAB Function3/2(alpha)
  Add/1 -> Scope2/1, Sum2/1
  Integrator Limited1/1 -> Sum/2  "q"
  PID Controller/1 -> Sum1/1, " Rate"/1, Scope3/1
  Sum1/1 -> Integrator Limited1/1  "q_dot"
  C1/1 -> Sum1/2
  Sum/1 -> Scope4/1, PID Controller/1
  q_des/1 -> Sum/1
  Demux/3 -> Add/3
  Demux/2 -> Add/2
  " Real Rates"/1 -> Product/2
  Demux/4 -> Add/4
  Demux/5 -> Add/5
  Demux/1 -> Add/1
  Product/1 -> Scope5/1, Demux/1
  Power/1 -> Equal/2
  Saturation/1 -> Equal/1
  Constant3/1 -> Power/1
  Random Number/1 -> Saturation/1
  Constant4/1 -> Power/2
  Equal/1 -> Sample and Hold/Trigger, Switch/2
  Product1/1 -> Product/1
  [delta_fault] -> Product1/2
  Constant2/1 -> Product1/1
  delta_fault/1 -> [delta_fault], MATLAB Function3/5(delta_fault)
  " "/1 -> Add/6
